simulink model "LMOL"  (R2024b)
settings: Solver=FixedStepAuto  StartTime=0  StopTime=inf  FixedStep=0.001  RelTol=1e-3  AbsTol=1e-6
values from neighbouring files (symbols this model uses):
  Ixx = 135582    [initialization.m]
  Iyy = 149140.0    (= 149140)    [initialization.m]
  Izz = 135582    [initialization.m]
undefined symbols (not defined in the file or in its folder): datetime, juliandate
Description:
  | Apollo Lunar Module Digital Autopilot
settings Model: RequirementInfo=9  SimulationMode=accelerator  Creator=The MathWorks, Inc.  LastModifiedBy=abdma
settings SolverCC: AutoScaleAbsTol=off  AlgebraicLoopSolver=TrustRegion  MaxZcPerStep=1
settings DataIOCC: SaveFormat=Array  ReturnWorkspaceOutputs=off  SignalLoggingName=logsOut
settings OptimizationCC: BlockReduction=off  ExpressionDepthLimit=2147483647  InitFltsAndDblsToZero=on
settings DebuggingCC: SaveWithParameterizedLinksMsg=none  SignalResolutionControl=TryResolveAllWithWarning  MultiTaskDSMMsg=warning  MultiTaskCondExecSysMsg=none  SigSpecEnsureSampleTimeMsg=none  FcnCallInpInsideContextMsg=warning  UnconnectedInputMsg=warning  UnconnectedOutputMsg=warning  UnconnectedLineMsg=warning  StateNameClashWarn=warning  SFUnexpectedBacktrackingDiag=warning  SFNoUnconditionalDefaultTransitionDiag=warning  SFExecutionAtInitializationDiag=none  ArithmeticOperatorsInVariantConditions=warning
settings HardwareCC: ProdBitPerPointer=32  ProdBitPerSizeT=32  ProdBitPerPtrDiffT=32  ProdLargestAtomicFloat=None  ProdIntDivRoundTo=Undefined  ProdEndianess=Unspecified  ProdWordSize=32  ProdHWDeviceType=Specified
settings ModelReferenceCC: EnableRefExpFcnMdlSchedulingChecks=on  PropagateSignalLabelsOutOfModel=off
settings SFSimCC: SimUseLocalCustomCode=off  SimParseCustomCode=off  CustomCodeUndefinedFunction=UseInterfaceOnly
settings RTWCC: RTWUseLocalCustomCode=off  GPUComputeCapability=3.5  DLArmComputeVersion=19.05
settings CodeAppCC: StateflowObjectComments=on
settings GRTTargetCC: TargetLangStandard=C89/C90 (ANSI)
settings ConfigComp: CovMetricSettings=d  CovSaveCumulativeToWorkspaceVar=on  CovSaveSingleToWorkspaceVar=on  CovExternalEMLEnable=off

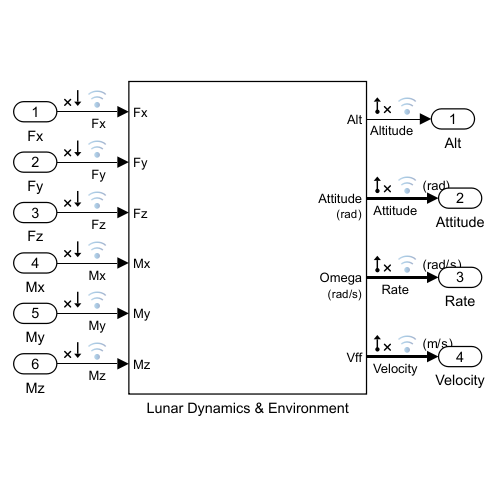
[thumbnail: Simulink's stored preview of the top-level diagram]
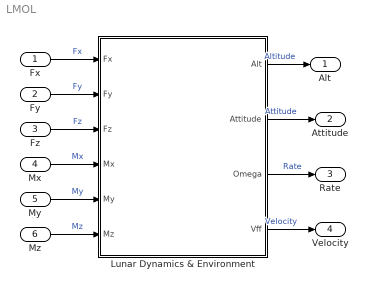
== system LMOL ==
  Fx : Inport
  Fy : Inport  Port=2
  Fz : Inport  Port=3
  Mx : Inport  Port=4
  My : Inport  Port=5
  Mz : Inport  Port=6
  Lunar Dynamics & Environment : Subsystem
  Alt : Outport
  Attitude : Outport  Port=2
  Rate : Outport  Port=3
  Velocity : Outport  Port=4
  wires:
  Mx/1 -> Lunar Dynamics & Environment/4(Mx)  "Mx"
  Lunar Dynamics & Environment/1(Alt) -> Alt/1  "Altitude"
  Lunar Dynamics & Environment/2(Attitude) -> Attitude/1  "Attitude"
  Lunar Dynamics & Environment/3(Omega) -> Rate/1  "Rate"
  Fz/1 -> Lunar Dynamics & Environment/3(Fz)  "Fz"
  My/1 -> Lunar Dynamics & Environment/5(My)  "My"
  Mz/1 -> Lunar Dynamics & Environment/6(Mz)  "Mz"
  Lunar Dynamics & Environment/4(Vff) -> Velocity/1  "Velocity"
  Fx/1 -> Lunar Dynamics & Environment/1(Fx)  "Fx"
  Fy/1 -> Lunar Dynamics & Environment/2(Fy)  "Fy"

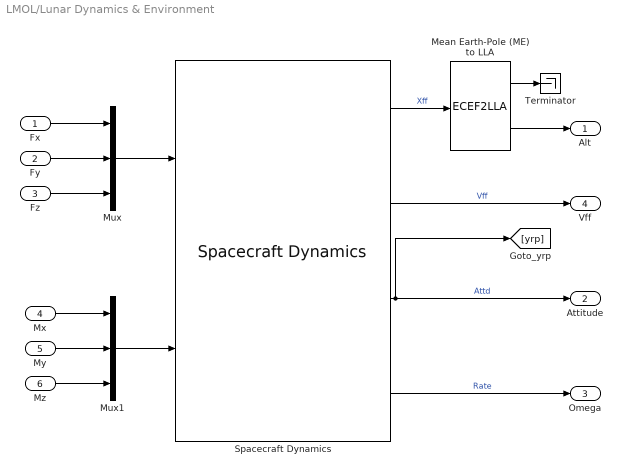
== system LMOL/Lunar Dynamics & Environment ==
  Fx : Inport
  Fy : Inport  Port=2
  Fz : Inport  Port=3
  Mx : Inport  Port=4
  My : Inport  Port=5
  Mz : Inport  Port=6
  Mean Earth-Pole (ME) to LLA : ECEF2LLA  ptype=Custom  F=0.0012  R=1737.4e3
  Mux : Mux  Inputs=3
  Mux1 : Mux  Inputs=3
  Spacecraft Dynamics : SpacecraftDynamics  accelFrame=Fixed-frame  outportFrame=Fixed-frame  startDate=juliandate(datetime('20-Jul-1969 19:08:44'))  dateOut=off  mass=mass  inertia=diag([Ixx,Iyy,Izz])  stateFormatNum=Fixed-frame state vector  inertialPosition=Xicrf0  inertialVelocity=Vicrf0  fixedPosition=Xff0  fixedVelocity=Vff0  attitudeFrame=NED  attitudeFormat=Euler angles  attitude=Att0  rotationOrder=XYZ  attitudeRate=Omg0  useGravGrad=off  centralBody=Moon  shDegree=60
      settings: AttributesFormatString=|
      | Central Body: %<centralBody>
      | Gravity Model: %<gravityModel> (%<moonSH>)
  Terminator : Terminator
  Alt : Outport  VectorParamsAs1DForOutWhenUnconnected=off
  Attitude : Outport  Port=2  Unit=rad  VectorParamsAs1DForOutWhenUnconnected=off
  Omega : Outport  Port=3  Unit=rad/s  VectorParamsAs1DForOutWhenUnconnected=off
  Vff : Outport  Port=4
  wires:
  Mean Earth-Pole (ME) to LLA/2 -> Alt/1
  Spacecraft Dynamics/1 -> Mean Earth-Pole (ME) to LLA/1  "Xff"
  Spacecraft Dynamics/3 -> Attitude/1, [yrp]  "Attd"
  Spacecraft Dynamics/4 -> Omega/1  "Rate"
  Mx/1 -> Mux1/1
  Mux1/1 -> Spacecraft Dynamics/2
  Mux/1 -> Spacecraft Dynamics/1
  Fx/1 -> Mux/1
  Fz/1 -> Mux/3
  My/1 -> Mux1/2
  Mz/1 -> Mux1/3
  Spacecraft Dynamics/2 -> Vff/1  "Vff"
  Fy/1 -> Mux/2
  Mean Earth-Pole (ME) to LLA/1 -> Terminator/1
